simulink model "powertrain_model"  (R2025a)
settings: Solver=ode23tb  StartTime=0.0  StopTime=simlength  FixedStep=tc  MaxStep=tc
values from neighbouring files (symbols this model uses):
  angle_error = angle_error_deg/180*pi    (= 0)    [init_model.m]
  CTRPIFF_CLIP_RELEASE = 0.001    [init_model.m]
  dead_time = dead_time_INV    (= 4.2e-07)    [init_model.m]
  dead_time_INV = 0.42e-6    (= 4.2e-07)    [init_model.m]
  DThs_init = 0    [init_model.m]
  emf_fb_p = 0.2    [init_model.m]
  emf_fb_p_ccaller_1 = emf_fb_p    (= 0.2)    [init_model.m]
  emf_fb_p_ccaller_2 = emf_fb_p    (= 0.2)    [init_model.m]
  emf_p = emf_fb_p*4/10    (= 0.08)    [init_model.m]
  emf_p_ccaller_1 = emf_fb_p_ccaller_1*4/10    (= 0.08)    [init_model.m]
  emf_p_ccaller_2 = emf_fb_p_ccaller_2*4/10    (= 0.08)    [init_model.m]
  fPWM_INV = 25e3    (= 25000)    [init_model.m]
  g0_reference_flt = fcut_reference_flt * ts_inv * 2*pi    (= 0.00100530964915)    [init_model.m]
  g1_reference_flt = 1 - g0_reference_flt    (= 0.998994690351)    [init_model.m]
  id_ref_if_pu = iload_rms_ref*sqrt(2)/ibez    [init_model.m]
  kalman_omega = kw    [init_model.m]
  kalman_theta = kg    [init_model.m]
  kg = K(1)    [init_model.m]
  ki_id = 2    [analysis_cc.m]    (also in init_model.m = 9)
  ki_iq = 9    [init_model.m]
  ki_w = 1    [init_model.m]
  kp_id = 0.15    [analysis_cc.m]    (also in init_model.m = 0.25)
  kp_iq = 0.2    [init_model.m]
  kp_w = 1    [init_model.m]
  kw = K(2)    [init_model.m]
  luenberger_l1 = Klo(1)    [init_model.m]
  luenberger_l2 = Klo(2)    [init_model.m]
  luenberger_l3 = Klo(3)    [init_model.m]
  motorc_m_scale = 2/3*Vdc_bez/ubez    [init_model.m]
  number_of_cells = 100    [init_model.m]
  omega_flt_fcut = 10    [init_model.m]
  omega_flt_g0 = omega_flt_fcut * ts_inv * 2*pi    (= 0.00251327412287)    [init_model.m]
  omega_flt_g1 = 1 - omega_flt_g0    (= 0.997486725877)    [init_model.m]
  omega_ref_if_pu = 1200*2*pi/omega_bez    [init_model.m]
  phase_compensation_omega = 0    [init_model.m]
  pwm_out_lim = 1    [init_model.m]
  Q = 10    [init_model.m]
  q1Kalman = ts_inv^2    (= 1.6e-09)    [init_model.m]
  q2Kalman = ts_inv^1    (= 4e-05)    [init_model.m]
  q3Kalman = 0    [init_model.m]
  rKalman = 1    [init_model.m]
  Tambient = 1    [init_model.m]
  tc = ts_inv/200    (= 2e-07)    [init_model.m]
  time_init = 0.025    [init_model.m]
  torque_ref = 64/ibez*torque_mode    [init_model.m]
  ts_inv = 1/fPWM_INV    (= 4e-05)    [init_model.m]
  tsample = ts_inv    (= 4e-05)    [init_model.m]
  u_flt_g0 = u_flt_fcut * ts_inv * 2*pi    (= 0.904778684234)    [init_model.m]
  u_flt_g1 = 1 - u_flt_g0    (= 0.0952213157661)    [init_model.m]
  Vdc_bez = 400    [init_model.m]
undefined symbols (not defined in the file or in its folder): b, ibez, Jm, Jm_norm, Ld_norm, Lq_norm, Ls_norm, magnitude, omega_bez, psi_bez, psi_m, psi_m_norm, R_RLload, Rload_eq, Rs_norm, tau_bez, weigth
libraries: fl_lib x100, nesl_utility x84, ee_lib x11, cstblocks x4, lithium_ion_cell_lib x1, simulink x1, pmsm_uvw_with_harmonics_lib x1, pmsm_spatial_harmonics_uvw_lib x1, flexshaft_lib x1
(part 2 of 6)

== system powertrain_model/inverter/MOS based inverter ==
  uab : Inport
  Demux : Demux  Outputs=6
  inverter : Subsystem
  sv_pwm : Subsystem
  threePhsModulator : Subsystem  Commented=on
  u : PMIOPort  Side=Left
  v : PMIOPort  Port=2  Side=Left
  w : PMIOPort  Port=3  Side=Left
  UDC(+) : PMIOPort  Port=4  Side=Right
  UDC(-) : PMIOPort  Port=5  Side=Right
  tag scope: gm1=global, gm2=global, gm3=global, gm4=global, gm5=global, gm6=global
  wires:
  Demux/6 -> [gm6]
  Demux/4 -> [gm4]
  Demux/5 -> [gm5]
  Demux/3 -> [gm3]
  Demux/1 -> [gm1]
  Demux/2 -> [gm2]
  sv_pwm/1(firing_gates) -> Demux/1
  uab/1 -> sv_pwm/1(ab), threePhsModulator/1(uab_pu)
  connections:
  inverter/LConn1 -- UDC(+)/RConn1
  inverter/LConn2 -- UDC(-)/RConn1
  v/RConn1 -- inverter/RConn2
  inverter/RConn1 -- u/RConn1
  inverter/RConn3 -- w/RConn1

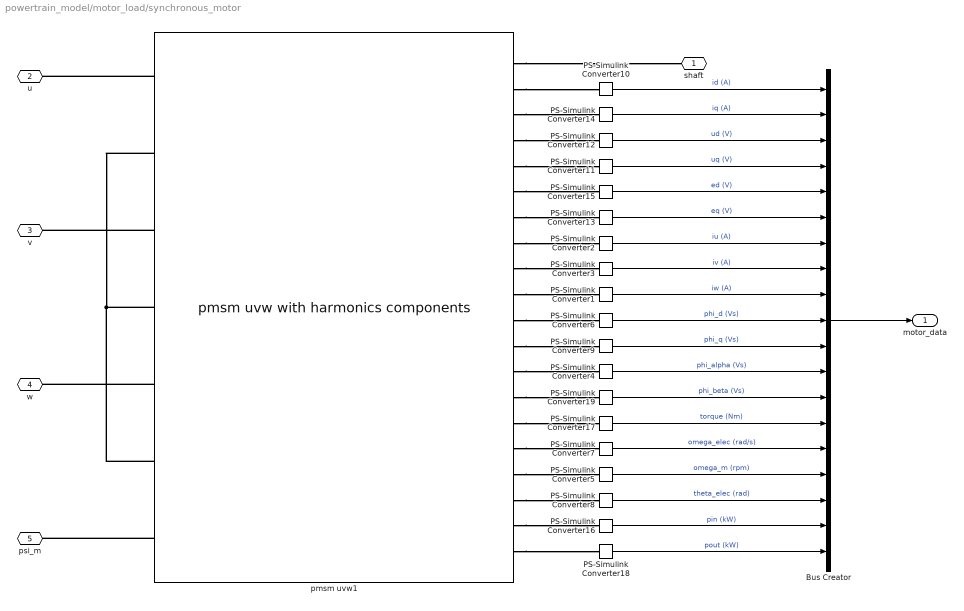
== system powertrain_model/motor_load/synchronous_motor ==
  Bus Creator : BusCreator  Inputs=19
  PS-Simulink Converter1 : nesl_utility/PS-Simulink Converter  PhysicalDomain=network_engine_domain  SubClassName=ps_output  LeftPortType=input  RightPortType=output  PseudoPeriodic=off  Frequencies=[]  VectorFormat=1-D array  Unit=A  AffineConversion=off
  PS-Simulink Converter10 : nesl_utility/PS-Simulink Converter  PhysicalDomain=network_engine_domain  SubClassName=ps_output  LeftPortType=input  RightPortType=output  PseudoPeriodic=off  Frequencies=[]  VectorFormat=1-D array  Unit=A  AffineConversion=on
  PS-Simulink Converter{11..13,15} (4 alike) : nesl_utility/PS-Simulink Converter  PhysicalDomain=network_engine_domain  SubClassName=ps_output  LeftPortType=input  RightPortType=output  PseudoPeriodic=off  Frequencies=[]  VectorFormat=1-D array  Unit=V  AffineConversion=on
  PS-Simulink Converter14 : nesl_utility/PS-Simulink Converter  PhysicalDomain=network_engine_domain  SubClassName=ps_output  LeftPortType=input  RightPortType=output  PseudoPeriodic=off  Frequencies=[]  VectorFormat=1-D array  Unit=A  AffineConversion=on
  PS-Simulink Converter16 : nesl_utility/PS-Simulink Converter  PhysicalDomain=network_engine_domain  SubClassName=ps_output  LeftPortType=input  RightPortType=output  PseudoPeriodic=off  Frequencies=[]  VectorFormat=1-D array  Unit=kW  AffineConversion=on
  PS-Simulink Converter17 : nesl_utility/PS-Simulink Converter  PhysicalDomain=network_engine_domain  SubClassName=ps_output  LeftPortType=input  RightPortType=output  PseudoPeriodic=off  Frequencies=[]  VectorFormat=1-D array  Unit=N*m  AffineConversion=on
  PS-Simulink Converter18 : nesl_utility/PS-Simulink Converter  PhysicalDomain=network_engine_domain  SubClassName=ps_output  LeftPortType=input  RightPortType=output  PseudoPeriodic=off  Frequencies=[]  VectorFormat=1-D array  Unit=kW  AffineConversion=on
  PS-Simulink Converter{4,6,9,19} (4 alike) : nesl_utility/PS-Simulink Converter  PhysicalDomain=network_engine_domain  SubClassName=ps_output  LeftPortType=input  RightPortType=output  PseudoPeriodic=off  Frequencies=[]  VectorFormat=1-D array  Unit=V*s  AffineConversion=on
  PS-Simulink Converter2 : nesl_utility/PS-Simulink Converter  PhysicalDomain=network_engine_domain  SubClassName=ps_output  LeftPortType=input  RightPortType=output  PseudoPeriodic=off  Frequencies=[]  VectorFormat=1-D array  Unit=A  AffineConversion=on
  PS-Simulink Converter3 : nesl_utility/PS-Simulink Converter  PhysicalDomain=network_engine_domain  SubClassName=ps_output  LeftPortType=input  RightPortType=output  PseudoPeriodic=off  Frequencies=[]  VectorFormat=1-D array  Unit=A  AffineConversion=off
  PS-Simulink Converter5 : nesl_utility/PS-Simulink Converter  PhysicalDomain=network_engine_domain  SubClassName=ps_output  LeftPortType=input  RightPortType=output  PseudoPeriodic=off  Frequencies=[]  VectorFormat=1-D array  Unit=rpm  AffineConversion=on
  PS-Simulink Converter7 : nesl_utility/PS-Simulink Converter  PhysicalDomain=network_engine_domain  SubClassName=ps_output  LeftPortType=input  RightPortType=output  PseudoPeriodic=off  Frequencies=[]  VectorFormat=1-D array  Unit=rad/s  AffineConversion=on
  PS-Simulink Converter8 : nesl_utility/PS-Simulink Converter  PhysicalDomain=network_engine_domain  SubClassName=ps_output  LeftPortType=input  RightPortType=output  PseudoPeriodic=off  Frequencies=[]  VectorFormat=1-D array  Unit=rad  AffineConversion=on
  pmsm uvw1 : pmsm_uvw_with_harmonics_lib/pmsm uvw with harmonics components  number_poles=number_poles  psi_m_p=psi_m V*s  Lmu=Lmu H  La=La H  Lb=Lb H  Rs=Rs Ohm  J=Jm kg*m^2  b=0 N*m*s/rad  b_square=0 N*m*s^2/rad^2  h5=4.0 percent  h7=1.0 percent  angle_error=0.5 rad  omega_specify=off  omega_priority=None  omega=0 rad/s  omega_nominal_specify=off  omega_nominal_unit=rad/s  omega_nominal_value=1  theta_specify=off  theta_priority=None  theta=0 rad  theta_nominal_specify=off  theta_nominal_unit=rad  theta_nominal_value=1  iu_specify=off  iu_priority=None  iu=0 A  iu_nominal_specify=off  iu_nominal_unit=A  iu_nominal_value=1  iv_specify=off  iv_priority=None  iv=0 A  iv_nominal_specify=off  iv_nominal_unit=A  iv_nominal_value=1  iw_specify=off  iw_priority=None  iw=0 A  iw_nominal_specify=off  iw_nominal_unit=A  iw_nominal_value=1  id_specify=off  id_priority=None  id=0 A  id_nominal_specify=off  id_nominal_unit=A  id_nominal_value=1  iq_specify=off  iq_priority=None  iq=0 A  iq_nominal_specify=off  iq_nominal_unit=A  iq_nominal_value=1  uv_specify=off  uv_priority=None  uv=0 V  uv_nominal_specify=off  uv_nominal_unit=V  uv_nominal_value=1  uu_specify=off  uu_priority=None  uu=0 V  uu_nominal_specify=off  uu_nominal_unit=V  uu_nominal_value=1  uw_specify=off  uw_priority=None  uw=0 V  uw_nominal_specify=off  uw_nominal_unit=V  uw_nominal_value=1  ud_specify=off  ud_priority=None  ud=0 V  ud_nominal_specify=off  ud_nominal_unit=V  ud_nominal_value=1  uq_specify=off  uq_priority=None  uq=0 V  uq_nominal_specify=off  uq_nominal_unit=V  uq_nominal_value=1  psi_r_u_specify=off  psi_r_u_priority=None  psi_r_u=0 V*s  psi_r_u_nominal_specify=off  psi_r_u_nominal_unit=V*s  psi_r_u_nominal_value=1  psi_r_v_specify=off  psi_r_v_priority=None  psi_r_v=0 V*s  psi_r_v_nominal_specify=off  psi_r_v_nominal_unit=V*s  psi_r_v_nominal_value=1  psi_r_w_specify=off  psi_r_w_priority=None  psi_r_w=0 V*s  psi_r_w_nominal_specify=off  psi_r_w_nominal_unit=V*s  psi_r_w_nominal_value=1  psi_s_d_specify=off  psi_s_d_priority=None  psi_s_d=0.0 V*s  psi_s_d_nominal_specify=off  psi_s_d_nominal_unit=V*s  psi_s_d_nominal_value=1  psi_s_q_specify=off  psi_s_q_priority=None  psi_s_q=0.0 V*s  psi_s_q_nominal_specify=off  psi_s_q_nominal_unit=V*s  psi_s_q_nominal_value=1  psi_r_d_specify=off  psi_r_d_priority=None  psi_r_d=0.0 V*s  psi_r_d_nominal_specify=off  psi_r_d_nominal_unit=V*s  psi_r_d_nominal_value=1  psi_r_q_specify=off  psi_r_q_priority=None  psi_r_q=0.0 V*s  psi_r_q_nominal_specify=off  psi_r_q_nominal_unit=V*s  psi_r_q_nominal_value=1  psi_r_alpha_specify=off  psi_r_alpha_priority=None  psi_r_alpha=0.0 V*s  psi_r_alpha_nominal_specify=off  psi_r_alpha_nominal_unit=V*s  psi_r_alpha_nominal_value=1  psi_r_beta_specify=off  psi_r_beta_priority=None  psi_r_beta=0.0 V*s  psi_r_beta_nominal_specify=off  psi_r_beta_nominal_unit=V*s  psi_r_beta_nominal_value=1  psi_s_alpha_specify=off  psi_s_alpha_priority=None  psi_s_alpha=0.0 V*s  psi_s_alpha_nominal_specify=off  psi_s_alpha_nominal_unit=V*s  psi_s_alpha_nominal_value=1  psi_s_beta_specify=off  psi_s_beta_priority=None  psi_s_beta=0.0 V*s  psi_s_beta_nominal_specify=off  psi_s_beta_nominal_unit=V*s  psi_s_beta_nominal_value=1  tau_l_specify=off  tau_l_priority=None  tau_l=0 N*m  tau_l_nominal_specify=off  tau_l_nominal_unit=N*m  tau_l_nominal_value=1  tau_m_specify=off  tau_m_priority=None  tau_m=0 N*m  tau_m_nominal_specify=off  tau_m_nominal_unit=N*m  tau_m_nominal_value=1
      settings: InternalSimscapePortConfiguration="{\"Bottom\":[],\"Left\":[{\"id\":\"uu_p\",\"label\":\"_uu+_\",\"type\":\"foundation.electrical.electrical\"},{\"id\":\"uu_n\",\"label\":\"_uu-_\",\"type\":\"foundation.electrical.electrical\"},{\"id\":\"uv_p\",\"label\":\"_uv+_\",\"type\":\"foundation.electrical.electrical\"},{\"id\":\"uv_n\",\"label\":\"_uv-_\",\"type\":\"foundation.electrical.electrical\"},{\"id\":\"uw_p\",\"label\":\"_uw+_\",\"type\":\"foundation.electrical.electrical\"},{\"id\":\"uw_n\",\"label\":\"_uw-_\",\"type\":\"foundation.electrical.electrical\"},{\"id\":\"psi_m\",\"label\":\"_psi_m_\",\"type\":\"input\"}],\"Right\":[{\"id\":\"S\",\"label\":\"_S_\",\"type\":\"foundation.mechanical.rotational.rotational\"},{\"id\":\"id_out\",\"label\":\"_id_\",\"type\":\"output\"},{\"id\":\"iq_out\",\"label\":\"_iq_\",\"type\":\"output\"},{\"id\":\"ud_out\",\"label\":\"_ud_\",\"type\":\"output\"},{\"id\":\"uq_out\",\"label\":\"_uq_\",\"type\":\"output\"},{\"id\":\"ed_out\",\"label\":\"_ed_\",\"type\":\"output\"},{\"id\":\"eq_out\",\"label\":\"_eq_\",\"type\":\"output\"},{\"id\":\"iu_out\",\"label\":\"_iu_\",\"type\":\"output\"},{\"id\":\"iv_out\",\"label\":\"_iv_\",\"type\":\"output\"},{\"id\":\"iw_out\",\"label\":\"_iw_\",\"type\":\"output\"},{\"id\":\"psi_r_d_out\",\"label\":\"_psi_r_d_\",\"type\":\"output\"},{\"id\":\"psi_r_q_out\",\"label\":\"_psi_r_q\",\"type\":\"output\"},{\"id\":\"psi_r_alpha_out\",\"label\":\"_psi_r_alpha_\",\"type\":\"output\"},{\"id\":\"psi_r_beta_out\",\"label\":\"_psi_r_beta\",\"type\":\"output\"},{\"id\":\"tau_out\",\"label\":\"_torque_\",\"type\":\"output\"},{\"id\":\"omega_out\",\"label\":\"_omega_elec_\",\"type\":\"output\"},{\"id\":\"omega_m_out\",\"label\":\"_omega_m_\",\"type\":\"output\"},{\"id\":\"theta_out\",\"label\":\"_theta_elec_\",\"type\":\"output\"},{\"id\":\"pin_out\",\"label\":\"_pin_\",\"type\":\"output\"},{\"id\":\"pout_out\",\"label\":\"_pout_\",\"type\":\"output\"}],\"Top\":[]}"
  shaft : PMIOPort  Side=Right
  u : PMIOPort  Port=2  Side=Left
  v : PMIOPort  Port=3  Side=Left
  w : PMIOPort  Port=4  Side=Left
  psi_m : PMIOPort  Port=5  Side=Left
  motor_data : Outport
  wires:
  PS-Simulink Converter10/1 -> Bus Creator/1  "id (A)"
  PS-Simulink Converter14/1 -> Bus Creator/2  "iq (A)"
  PS-Simulink Converter12/1 -> Bus Creator/3  "ud (V)"
  PS-Simulink Converter11/1 -> Bus Creator/4  "uq (V)"
  PS-Simulink Converter15/1 -> Bus Creator/5  "ed (V)"
  PS-Simulink Converter13/1 -> Bus Creator/6  "eq (V)"
  PS-Simulink Converter2/1 -> Bus Creator/7  "iu (A)"
  PS-Simulink Converter3/1 -> Bus Creator/8  "iv (A)"
  PS-Simulink Converter1/1 -> Bus Creator/9  "iw (A)"
  PS-Simulink Converter6/1 -> Bus Creator/10  "phi_d (Vs)"
  PS-Simulink Converter9/1 -> Bus Creator/11  "phi_q (Vs)"
  Bus Creator/1 -> motor_data/1
  PS-Simulink Converter18/1 -> Bus Creator/19  "pout (kW)"
  PS-Simulink Converter16/1 -> Bus Creator/18  "pin (kW)"
  PS-Simulink Converter8/1 -> Bus Creator/17  "theta_elec (rad)"
  PS-Simulink Converter5/1 -> Bus Creator/16  "omega_m (rpm)"
  PS-Simulink Converter7/1 -> Bus Creator/15  "omega_elec (rad/s)"
  PS-Simulink Converter17/1 -> Bus Creator/14  "torque (Nm)"
  PS-Simulink Converter4/1 -> Bus Creator/12  "phi_alpha (Vs)"
  PS-Simulink Converter19/1 -> Bus Creator/13  "phi_beta (Vs)"
  connections:
  pmsm uvw1/RConn8 -- PS-Simulink Converter2/LConn1
  pmsm uvw1/RConn9 -- PS-Simulink Converter3/LConn1
  pmsm uvw1/RConn3 -- PS-Simulink Converter14/LConn1
  pmsm uvw1/RConn4 -- PS-Simulink Converter12/LConn1
  pmsm uvw1/RConn2 -- PS-Simulink Converter10/LConn1
  pmsm uvw1/LConn2 -- pmsm uvw1/LConn6 -- pmsm uvw1/LConn4
  pmsm uvw1/RConn7 -- PS-Simulink Converter13/LConn1
  pmsm uvw1/LConn1 -- u/RConn1
  pmsm uvw1/RConn12 -- PS-Simulink Converter9/LConn1
  pmsm uvw1/RConn10 -- PS-Simulink Converter1/LConn1
  pmsm uvw1/LConn5 -- w/RConn1
  pmsm uvw1/LConn7 -- psi_m/RConn1
  pmsm uvw1/RConn5 -- PS-Simulink Converter11/LConn1
  pmsm uvw1/RConn11 -- PS-Simulink Converter6/LConn1
  pmsm uvw1/RConn6 -- PS-Simulink Converter15/LConn1
  pmsm uvw1/LConn3 -- v/RConn1
  pmsm uvw1/RConn1 -- shaft/RConn1
  pmsm uvw1/RConn15 -- PS-Simulink Converter17/LConn1
  pmsm uvw1/RConn16 -- PS-Simulink Converter7/LConn1
  pmsm uvw1/RConn17 -- PS-Simulink Converter5/LConn1
  pmsm uvw1/RConn18 -- PS-Simulink Converter8/LConn1
  pmsm uvw1/RConn19 -- PS-Simulink Converter16/LConn1
  pmsm uvw1/RConn20 -- PS-Simulink Converter18/LConn1
  pmsm uvw1/RConn13 -- PS-Simulink Converter4/LConn1
  pmsm uvw1/RConn14 -- PS-Simulink Converter19/LConn1

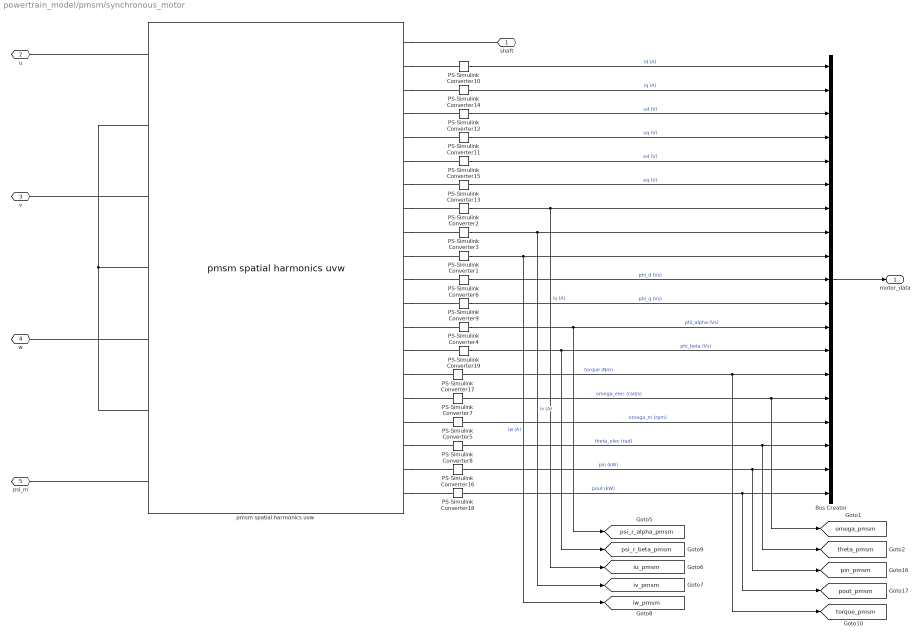
== system powertrain_model/pmsm/synchronous_motor ==
  Bus Creator : BusCreator  Inputs=19
  PS-Simulink Converter{1..3,10,14} (5 alike) : nesl_utility/PS-Simulink Converter  PhysicalDomain=network_engine_domain  SubClassName=ps_output  LeftPortType=input  RightPortType=output  PseudoPeriodic=off  Frequencies=[]  VectorFormat=1-D array  Unit=A  AffineConversion=on
  PS-Simulink Converter{11..13,15} (4 alike) : nesl_utility/PS-Simulink Converter  PhysicalDomain=network_engine_domain  SubClassName=ps_output  LeftPortType=input  RightPortType=output  PseudoPeriodic=off  Frequencies=[]  VectorFormat=1-D array  Unit=V  AffineConversion=on
  PS-Simulink Converter16 : nesl_utility/PS-Simulink Converter  PhysicalDomain=network_engine_domain  SubClassName=ps_output  LeftPortType=input  RightPortType=output  PseudoPeriodic=off  Frequencies=[]  VectorFormat=1-D array  Unit=kW  AffineConversion=on
  PS-Simulink Converter17 : nesl_utility/PS-Simulink Converter  PhysicalDomain=network_engine_domain  SubClassName=ps_output  LeftPortType=input  RightPortType=output  PseudoPeriodic=off  Frequencies=[]  VectorFormat=1-D array  Unit=N*m  AffineConversion=on
  PS-Simulink Converter18 : nesl_utility/PS-Simulink Converter  PhysicalDomain=network_engine_domain  SubClassName=ps_output  LeftPortType=input  RightPortType=output  PseudoPeriodic=off  Frequencies=[]  VectorFormat=1-D array  Unit=kW  AffineConversion=on
  PS-Simulink Converter{4,6,9,19} (4 alike) : nesl_utility/PS-Simulink Converter  PhysicalDomain=network_engine_domain  SubClassName=ps_output  LeftPortType=input  RightPortType=output  PseudoPeriodic=off  Frequencies=[]  VectorFormat=1-D array  Unit=V*s  AffineConversion=on
  PS-Simulink Converter5 : nesl_utility/PS-Simulink Converter  PhysicalDomain=network_engine_domain  SubClassName=ps_output  LeftPortType=input  RightPortType=output  PseudoPeriodic=off  Frequencies=[]  VectorFormat=1-D array  Unit=rpm  AffineConversion=on
  PS-Simulink Converter7 : nesl_utility/PS-Simulink Converter  PhysicalDomain=network_engine_domain  SubClassName=ps_output  LeftPortType=input  RightPortType=output  PseudoPeriodic=off  Frequencies=[]  VectorFormat=1-D array  Unit=rad/s  AffineConversion=on
  PS-Simulink Converter8 : nesl_utility/PS-Simulink Converter  PhysicalDomain=network_engine_domain  SubClassName=ps_output  LeftPortType=input  RightPortType=output  PseudoPeriodic=off  Frequencies=[]  VectorFormat=1-D array  Unit=rad  AffineConversion=on
  pmsm spatial harmonics uvw : pmsm_spatial_harmonics_uvw_lib/pmsm spatial harmonics uvw  number_poles=number_poles  psi_m_p=psi_m V*s  Lmu=Lmu H  La=La H  Lb=Lb H  Rs=Rs Ohm  J=Jm kg*m^2  b=b N*m/(rad/s)  b_square=0 N*m*s^2/rad^2  h5=0 %h5_psm_percent percent  h7=0 %h7_psm_percent percent  omega_specify=off  omega_priority=None  omega=0 rad/s  omega_nominal_specify=off  omega_nominal_unit=rad/s  omega_nominal_value=1  theta_specify=off  theta_priority=None  theta=0 rad  theta_nominal_specify=off  theta_nominal_unit=rad  theta_nominal_value=1  iu_specify=off  iu_priority=None  iu=0 A  iu_nominal_specify=off  iu_nominal_unit=A  iu_nominal_value=1  iv_specify=off  iv_priority=None  iv=0 A  iv_nominal_specify=off  iv_nominal_unit=A  iv_nominal_value=1  iw_specify=off  iw_priority=None  iw=0 A  iw_nominal_specify=off  iw_nominal_unit=A  iw_nominal_value=1  id_specify=off  id_priority=None  id=0 A  id_nominal_specify=off  id_nominal_unit=A  id_nominal_value=1  iq_specify=off  iq_priority=None  iq=0 A  iq_nominal_specify=off  iq_nominal_unit=A  iq_nominal_value=1  uv_specify=off  uv_priority=None  uv=0 V  uv_nominal_specify=off  uv_nominal_unit=V  uv_nominal_value=1  uu_specify=off  uu_priority=None  uu=0 V  uu_nominal_specify=off  uu_nominal_unit=V  uu_nominal_value=1  uw_specify=off  uw_priority=None  uw=0 V  uw_nominal_specify=off  uw_nominal_unit=V  uw_nominal_value=1  ud_specify=off  ud_priority=None  ud=0 V  ud_nominal_specify=off  ud_nominal_unit=V  ud_nominal_value=1  uq_specify=off  uq_priority=None  uq=0 V  uq_nominal_specify=off  uq_nominal_unit=V  uq_nominal_value=1  psi_r_u_specify=off  psi_r_u_priority=None  psi_r_u=0 V*s  psi_r_u_nominal_specify=off  psi_r_u_nominal_unit=V*s  psi_r_u_nominal_value=1  psi_r_v_specify=off  psi_r_v_priority=None  psi_r_v=0 V*s  psi_r_v_nominal_specify=off  psi_r_v_nominal_unit=V*s  psi_r_v_nominal_value=1  psi_r_w_specify=off  psi_r_w_priority=None  psi_r_w=0 V*s  psi_r_w_nominal_specify=off  psi_r_w_nominal_unit=V*s  psi_r_w_nominal_value=1  psi_s_d_specify=off  psi_s_d_priority=None  psi_s_d=0.0 V*s  psi_s_d_nominal_specify=off  psi_s_d_nominal_unit=V*s  psi_s_d_nominal_value=1  psi_s_q_specify=off  psi_s_q_priority=None  psi_s_q=0.0 V*s  psi_s_q_nominal_specify=off  psi_s_q_nominal_unit=V*s  psi_s_q_nominal_value=1  psi_r_d_specify=off  psi_r_d_priority=None  psi_r_d=0.0 V*s  psi_r_d_nominal_specify=off  psi_r_d_nominal_unit=V*s  psi_r_d_nominal_value=1  psi_r_q_specify=off  psi_r_q_priority=None  psi_r_q=0.0 V*s  psi_r_q_nominal_specify=off  psi_r_q_nominal_unit=V*s  psi_r_q_nominal_value=1  psi_r_alpha_specify=on  psi_r_alpha_priority=High  psi_r_alpha=psi_m V*s  psi_r_alpha_nominal_specify=off  psi_r_alpha_nominal_unit=V*s  psi_r_alpha_nominal_value=1  psi_r_beta_specify=on  psi_r_beta_priority=High  psi_r_beta=0.0 V*s  psi_r_beta_nominal_specify=off  psi_r_beta_nominal_unit=V*s  psi_r_beta_nominal_value=1  psi_s_alpha_specify=on  psi_s_alpha_priority=High  psi_s_alpha=psi_m V*s  psi_s_alpha_nominal_specify=off  psi_s_alpha_nominal_unit=V*s  psi_s_alpha_nominal_value=1  psi_s_beta_specify=on  psi_s_beta_priority=High  psi_s_beta=0.0 V*s  psi_s_beta_nominal_specify=off  psi_s_beta_nominal_unit=V*s  psi_s_beta_nominal_value=1  tau_l_specify=off  tau_l_priority=None  tau_l=0 N*m  tau_l_nominal_specify=off  tau_l_nominal_unit=N*m  tau_l_nominal_value=1  tau_m_specify=off  tau_m_priority=None  tau_m=0 N*m  tau_m_nominal_specify=off  tau_m_nominal_unit=N*m  tau_m_nominal_value=1
      settings: InternalSimscapePortConfiguration="{\"Bottom\":[],\"Left\":[{\"id\":\"uu_p\",\"label\":\"_uu+_\",\"type\":\"foundation.electrical.electrical\"},{\"id\":\"uu_n\",\"label\":\"_uu-_\",\"type\":\"foundation.electrical.electrical\"},{\"id\":\"uv_p\",\"label\":\"_uv+_\",\"type\":\"foundation.electrical.electrical\"},{\"id\":\"uv_n\",\"label\":\"_uv-_\",\"type\":\"foundation.electrical.electrical\"},{\"id\":\"uw_p\",\"label\":\"_uw+_\",\"type\":\"foundation.electrical.electrical\"},{\"id\":\"uw_n\",\"label\":\"_uw-_\",\"type\":\"foundation.electrical.electrical\"},{\"id\":\"psi_m\",\"label\":\"_psi_m_\",\"type\":\"input\"}],\"Right\":[{\"id\":\"S\",\"label\":\"_S_\",\"type\":\"foundation.mechanical.rotational.rotational\"},{\"id\":\"id_out\",\"label\":\"_id_\",\"type\":\"output\"},{\"id\":\"iq_out\",\"label\":\"_iq_\",\"type\":\"output\"},{\"id\":\"ud_out\",\"label\":\"_ud_\",\"type\":\"output\"},{\"id\":\"uq_out\",\"label\":\"_uq_\",\"type\":\"output\"},{\"id\":\"ed_out\",\"label\":\"_ed_\",\"type\":\"output\"},{\"id\":\"eq_out\",\"label\":\"_eq_\",\"type\":\"output\"},{\"id\":\"iu_out\",\"label\":\"_iu_\",\"type\":\"output\"},{\"id\":\"iv_out\",\"label\":\"_iv_\",\"type\":\"output\"},{\"id\":\"iw_out\",\"label\":\"_iw_\",\"type\":\"output\"},{\"id\":\"psi_r_d_out\",\"label\":\"_psi_r_d_\",\"type\":\"output\"},{\"id\":\"psi_r_q_out\",\"label\":\"_psi_r_q\",\"type\":\"output\"},{\"id\":\"psi_r_alpha_out\",\"label\":\"_psi_r_alpha_\",\"type\":\"output\"},{\"id\":\"psi_r_beta_out\",\"label\":\"_psi_r_beta\",\"type\":\"output\"},{\"id\":\"tau_out\",\"label\":\"_torque_\",\"type\":\"output\"},{\"id\":\"omega_out\",\"label\":\"_omega_elec_\",\"type\":\"output\"},{\"id\":\"omega_m_out\",\"label\":\"_omega_m_\",\"type\":\"output\"},{\"id\":\"theta_out\",\"label\":\"_theta_elec_\",\"type\":\"output\"},{\"id\":\"pin_out\",\"label\":\"_pin_\",\"type\":\"output\"},{\"id\":\"pout_out\",\"label\":\"_pout_\",\"type\":\"output\"}],\"Top\":[]}"
  shaft : PMIOPort  Side=Right
  u : PMIOPort  Port=2  Side=Left
  v : PMIOPort  Port=3  Side=Left
  w : PMIOPort  Port=4  Side=Left
  psi_m : PMIOPort  Port=5  Side=Left
  motor_data : Outport
  tag scope: iu_pmsm=global, iv_pmsm=global, iw_pmsm=global, omega_pmsm=global, pin_pmsm=global, pout_pmsm=global, psi_r_alpha_pmsm=global, psi_r_beta_pmsm=global, theta_pmsm=global, torque_pmsm=global
  wires:
  PS-Simulink Converter10/1 -> Bus Creator/1  "id (A)"
  PS-Simulink Converter14/1 -> Bus Creator/2  "iq (A)"
  PS-Simulink Converter12/1 -> Bus Creator/3  "ud (V)"
  PS-Simulink Converter11/1 -> Bus Creator/4  "uq (V)"
  PS-Simulink Converter15/1 -> Bus Creator/5  "ed (V)"
  PS-Simulink Converter13/1 -> Bus Creator/6  "eq (V)"
  PS-Simulink Converter2/1 -> Bus Creator/7, [iu_pmsm]  "iu (A)"
  PS-Simulink Converter3/1 -> Bus Creator/8, [iv_pmsm]  "iv (A)"
  PS-Simulink Converter1/1 -> Bus Creator/9, [iw_pmsm]  "iw (A)"
  PS-Simulink Converter6/1 -> Bus Creator/10  "phi_d (Vs)"
  PS-Simulink Converter9/1 -> Bus Creator/11  "phi_q (Vs)"
  Bus Creator/1 -> motor_data/1
  PS-Simulink Converter18/1 -> [pout_pmsm], Bus Creator/19  "pout (kW)"
  PS-Simulink Converter16/1 -> [pin_pmsm], Bus Creator/18  "pin (kW)"
  PS-Simulink Converter8/1 -> [theta_pmsm], Bus Creator/17  "theta_elec (rad)"
  PS-Simulink Converter5/1 -> Bus Creator/16  "omega_m (rpm)"
  PS-Simulink Converter7/1 -> [omega_pmsm], Bus Creator/15  "omega_elec (rad/s)"
  PS-Simulink Converter17/1 -> [torque_pmsm], Bus Creator/14  "torque (Nm)"
  PS-Simulink Converter4/1 -> Bus Creator/12, [psi_r_alpha_pmsm]  "phi_alpha (Vs)"
  PS-Simulink Converter19/1 -> Bus Creator/13, [psi_r_beta_pmsm]  "phi_beta (Vs)"
  connections:
  pmsm spatial harmonics uvw/RConn8 -- PS-Simulink Converter2/LConn1
  pmsm spatial harmonics uvw/RConn9 -- PS-Simulink Converter3/LConn1
  pmsm spatial harmonics uvw/RConn3 -- PS-Simulink Converter14/LConn1
  pmsm spatial harmonics uvw/RConn4 -- PS-Simulink Converter12/LConn1
  pmsm spatial harmonics uvw/RConn2 -- PS-Simulink Converter10/LConn1
  pmsm spatial harmonics uvw/LConn2 -- pmsm spatial harmonics uvw/LConn6 -- pmsm spatial harmonics uvw/LConn4
  pmsm spatial harmonics uvw/RConn7 -- PS-Simulink Converter13/LConn1
  pmsm spatial harmonics uvw/LConn1 -- u/RConn1
  pmsm spatial harmonics uvw/RConn12 -- PS-Simulink Converter9/LConn1
  pmsm spatial harmonics uvw/RConn10 -- PS-Simulink Converter1/LConn1
  pmsm spatial harmonics uvw/LConn5 -- w/RConn1
  pmsm spatial harmonics uvw/LConn7 -- psi_m/RConn1
  pmsm spatial harmonics uvw/RConn5 -- PS-Simulink Converter11/LConn1
  pmsm spatial harmonics uvw/RConn11 -- PS-Simulink Converter6/LConn1
  pmsm spatial harmonics uvw/RConn6 -- PS-Simulink Converter15/LConn1
  pmsm spatial harmonics uvw/LConn3 -- v/RConn1
  pmsm spatial harmonics uvw/RConn1 -- shaft/RConn1
  pmsm spatial harmonics uvw/RConn15 -- PS-Simulink Converter17/LConn1
  pmsm spatial harmonics uvw/RConn16 -- PS-Simulink Converter7/LConn1
  pmsm spatial harmonics uvw/RConn17 -- PS-Simulink Converter5/LConn1
  pmsm spatial harmonics uvw/RConn18 -- PS-Simulink Converter8/LConn1
  pmsm spatial harmonics uvw/RConn19 -- PS-Simulink Converter16/LConn1
  pmsm spatial harmonics uvw/RConn20 -- PS-Simulink Converter18/LConn1
  pmsm spatial harmonics uvw/RConn13 -- PS-Simulink Converter4/LConn1
  pmsm spatial harmonics uvw/RConn14 -- PS-Simulink Converter19/LConn1

== system powertrain_model/propeller/Subsystem ==
  flexible shaft : flexshaft_lib/flexible shaft  b1=0 N*m*s/rad  J1=1e-4 kg*m^2  b2=0 N*m*s/rad  J2=1e-4 kg*m^2  b_theta=0 N*m*s/rad  k_theta=1e12 N*m/rad  w_1_specify=off  w_1_priority=None  w_1=0 rad/s  w_1_nominal_specify=off  w_1_nominal_value=1  w_1_nominal_unit=rad/s  w_2_specify=off  w_2_priority=None  w_2=0 rad/s  w_2_nominal_specify=off  w_2_nominal_value=1  w_2_nominal_unit=rad/s  t_1_specify=off  t_1_priority=None  t_1=0 N*m  t_1_nominal_specify=off  t_1_nominal_value=1  t_1_nominal_unit=N*m  t_2_specify=off  t_2_priority=None  t_2=0 N*m  t_2_nominal_specify=off  t_2_nominal_value=1  t_2_nominal_unit=N*m  t_theta_specify=off  t_theta_priority=None  t_theta=0 N*m  t_theta_nominal_specify=off  t_theta_nominal_value=1  t_theta_nominal_unit=N*m
      settings: InternalSimscapePortConfiguration="{\"Bottom\":[],\"Left\":[{\"id\":\"S1\",\"label\":\"S1\",\"type\":\"foundation.mechanical.rotational.rotational\"}],\"Right\":[{\"id\":\"S2\",\"label\":\"S2\",\"type\":\"foundation.mechanical.rotational.rotational\"}],\"Top\":[]}"
  s2 : PMIOPort  Side=Right
  s1 : PMIOPort  Port=2  Side=Left
  connections:
  flexible shaft/RConn1 -- s2/RConn1
  flexible shaft/LConn1 -- s1/RConn1

== system powertrain_model/battery_system/battery_system/LithiumIonBattery ==
  Current Sensor : fl_lib/Electrical/Electrical Sensors/Current Sensor
  Electrical Reference1 : fl_lib/Electrical/Electrical Elements/Electrical Reference
  PS-Simulink Converter4 : nesl_utility/PS-Simulink Converter  PhysicalDomain=network_engine_domain  SubClassName=ps_output  LeftPortType=input  RightPortType=output  PseudoPeriodic=off  Frequencies=[]  VectorFormat=1-D array  Unit=1  AffineConversion=off
  PS-Simulink Converter5 : nesl_utility/PS-Simulink Converter  PhysicalDomain=network_engine_domain  SubClassName=ps_output  LeftPortType=input  RightPortType=output  PseudoPeriodic=off  Frequencies=[]  VectorFormat=1-D array  Unit=V  AffineConversion=on
  SOC_estimator : Subsystem
  To Workspace1 : ToWorkspace  VariableName=idc_battery_sim  SampleTime=tc
      settings: MaxDataPoints=Nc
  To Workspace2 : ToWorkspace  VariableName=udc_battery_sim  SampleTime=tc
      settings: MaxDataPoints=Nc
  Unit Delay5 : UnitDelay  SampleTime=tsample  HasFrameUpgradeWarning=on
  Voltage Sensor : fl_lib/Electrical/Electrical Sensors/Voltage Sensor
  ibat/vdc : Scope  Commented=on  NumInputPorts=2
      settings: SampleTime=tsample  ActiveDisplayYMinimum=-422.32966  ActiveDisplayYMaximum=499.01489  DataLoggingVariableName=ScopeData6
  lithium ion cell analytical ocv : Subsystem
  Uout+ : PMIOPort  Side=Right
  Uout- : PMIOPort  Port=2  Side=Right
  wires:
  PS-Simulink Converter5/1 -> Unit Delay5/1
  PS-Simulink Converter4/1 -> To Workspace1/1, ibat/vdc/1  "i batt"
  Unit Delay5/1 -> To Workspace2/1, [vdc]
  [vdc] -> ibat/vdc/2  "vdc"
  connections:
  Current Sensor/RConn1 -- PS-Simulink Converter4/LConn1
  Uout+/RConn1 -- Current Sensor/RConn2 -- Voltage Sensor/LConn1
  Voltage Sensor/RConn1 -- PS-Simulink Converter5/LConn1
  Voltage Sensor/RConn2 -- Electrical Reference1/LConn1 -- lithium ion cell analytical ocv/RConn2 -- Uout-/RConn1
  lithium ion cell analytical ocv/RConn1 -- Current Sensor/LConn1

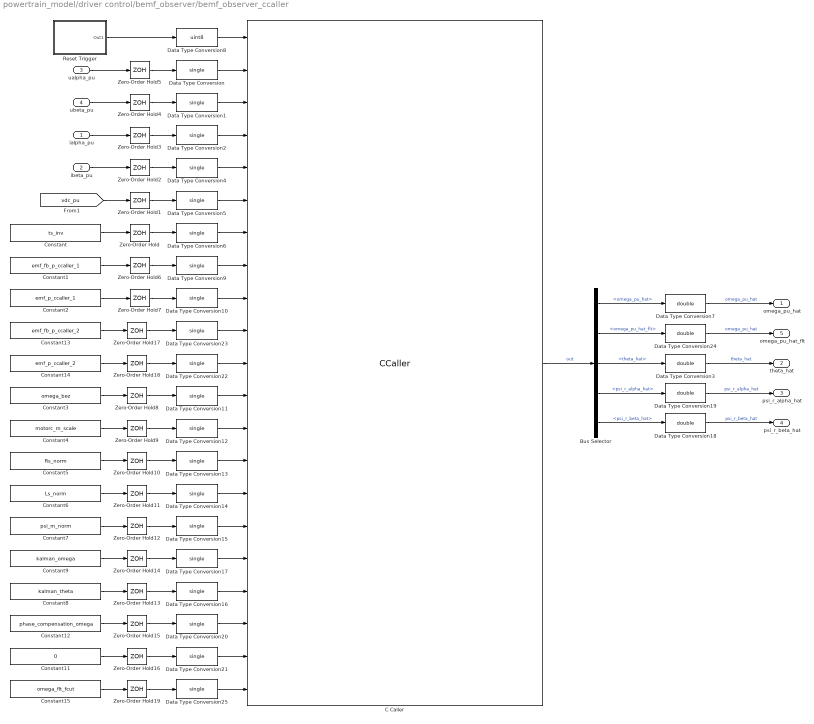
== system powertrain_model/driver control/bemf_observer/bemf_observer_ccaller ==
  ialpha_pu : Inport
  ibeta_pu : Inport  Port=2
  ualpha_pu : Inport  Port=3
  ubeta_pu : Inport  Port=4
  Bus Selector : BusSelector  OutputSignals=omega_pu_hat,omega_pu_hat_flt,theta_hat,psi_r_alpha_hat,psi_r_beta_hat
  C Caller : CCaller  FunctionName=bemf_obsv_process_simulink  PortSpecificationStruct="%)30     .    N\"8   8    (     @         %    \"    !8    !     0         %  0 \"0    $    _    07)G3F%M90  4&]R=$YA;64 4V-O<&4     26YD97@     5'EP90      4VEZ90      27-';&]B86P   X    P    !@    @    $          4    (     0    ,    !         !   P!O=70 #@   #     &    \"     0         !0    @    !     P    $         $  # &]U=  .    .     8    (    !          %    \"     $    &     0         0  ...(+12985 chars)"  SampleTime=ts_inv
  Constant : Constant  Value=ts_inv
  Constant1 : Constant  Value=emf_fb_p_ccaller_1
  Constant11 : Constant  Value=0
  Constant12 : Constant  Value=phase_compensation_omega  VectorParams1D=off
  Constant13 : Constant  Value=emf_fb_p_ccaller_2
  Constant14 : Constant  Value=emf_p_ccaller_2
  Constant15 : Constant  Value=omega_flt_fcut
  Constant2 : Constant  Value=emf_p_ccaller_1
  Constant3 : Constant  Value=omega_bez
  Constant4 : Constant  Value=motorc_m_scale
  Constant5 : Constant  Value=Rs_norm
  Constant6 : Constant  Value=Ls_norm
  Constant7 : Constant  Value=psi_m_norm
  Constant8 : Constant  Value=kalman_theta
  Constant9 : Constant  Value=kalman_omega
  Data Type Conversion{,1..2,4..6,9..17,20..23,25} (20 alike) : DataTypeConversion  OutDataTypeStr=single  SaturateOnIntegerOverflow=off  RndMeth=Floor
  Data Type Conversion{3,7,18..19,24} (5 alike) : DataTypeConversion  OutDataTypeStr=double  SaturateOnIntegerOverflow=off  RndMeth=Floor
  Data Type Conversion8 : DataTypeConversion  OutDataTypeStr=uint8  SaturateOnIntegerOverflow=off  RndMeth=Floor
  Reset Trigger : Subsystem
  Zero-Order Hold{,1..19} (20 alike) : ZeroOrderHold  SampleTime=ts_inv
  omega_pu_hat : Outport
  theta_hat : Outport  Port=2
  psi_r_alpha_hat : Outport  Port=3
  psi_r_beta_hat : Outport  Port=4
  omega_pu_hat_flt : Outport  Port=5
  wires:
  Bus Selector/1 -> Data Type Conversion7/1  "<omega_pu_hat>"
  Bus Selector/2 -> Data Type Conversion24/1  "<omega_pu_hat_flt>"
  Bus Selector/3 -> Data Type Conversion3/1  "<theta_hat>"
  Bus Selector/4 -> Data Type Conversion19/1  "<psi_r_alpha_hat>"
  Bus Selector/5 -> Data Type Conversion18/1  "<psi_r_beta_hat>"
  Zero-Order Hold19/1 -> Data Type Conversion25/1
  Constant15/1 -> Zero-Order Hold19/1
  Data Type Conversion24/1 -> omega_pu_hat_flt/1  "omega_pu_hat"
  Zero-Order Hold17/1 -> Data Type Conversion23/1
  Zero-Order Hold18/1 -> Data Type Conversion22/1
  Constant13/1 -> Zero-Order Hold17/1
  Constant14/1 -> Zero-Order Hold18/1
  Constant11/1 -> Zero-Order Hold16/1
  Zero-Order Hold16/1 -> Data Type Conversion21/1
  Zero-Order Hold15/1 -> Data Type Conversion20/1
  Constant12/1 -> Zero-Order Hold15/1
  Constant2/1 -> Zero-Order Hold7/1
  Constant1/1 -> Zero-Order Hold6/1
  Data Type Conversion18/1 -> psi_r_beta_hat/1  "psi_r_beta_hat"
  Data Type Conversion19/1 -> psi_r_alpha_hat/1  "psi_r_alpha_hat"
  Data Type Conversion3/1 -> theta_hat/1  "theta_hat"
  Data Type Conversion7/1 -> omega_pu_hat/1  "omega_pu_hat"
  C Caller/1 -> Bus Selector/1  "out"
  Constant7/1 -> Zero-Order Hold12/1
  Constant6/1 -> Zero-Order Hold11/1
  Constant9/1 -> Zero-Order Hold14/1
  Constant8/1 -> Zero-Order Hold13/1
  Constant5/1 -> Zero-Order Hold10/1
  Constant4/1 -> Zero-Order Hold9/1
  Constant3/1 -> Zero-Order Hold8/1
  Zero-Order Hold14/1 -> Data Type Conversion17/1
  Zero-Order Hold13/1 -> Data Type Conversion16/1
  Zero-Order Hold12/1 -> Data Type Conversion15/1
  Zero-Order Hold11/1 -> Data Type Conversion14/1
  Zero-Order Hold10/1 -> Data Type Conversion13/1
  Zero-Order Hold9/1 -> Data Type Conversion12/1
  Zero-Order Hold8/1 -> Data Type Conversion11/1
  Zero-Order Hold7/1 -> Data Type Conversion10/1
  Zero-Order Hold6/1 -> Data Type Conversion9/1
  Reset Trigger/1(Out1) -> Data Type Conversion8/1
  ibeta_pu/1 -> Zero-Order Hold2/1
  ubeta_pu/1 -> Zero-Order Hold4/1
  ialpha_pu/1 -> Zero-Order Hold3/1
  ualpha_pu/1 -> Zero-Order Hold5/1
  Constant/1 -> Zero-Order Hold/1
  [vdc_pu] -> Zero-Order Hold1/1
  Zero-Order Hold1/1 -> Data Type Conversion5/1
  Zero-Order Hold2/1 -> Data Type Conversion4/1
  Zero-Order Hold3/1 -> Data Type Conversion2/1
  Zero-Order Hold4/1 -> Data Type Conversion1/1
  Zero-Order Hold5/1 -> Data Type Conversion/1
  Zero-Order Hold/1 -> Data Type Conversion6/1
  Data Type Conversion/1 -> C Caller/2
  Data Type Conversion8/1 -> C Caller/1
  Data Type Conversion1/1 -> C Caller/3
  Data Type Conversion2/1 -> C Caller/4
  Data Type Conversion4/1 -> C Caller/5
  Data Type Conversion5/1 -> C Caller/6
  Data Type Conversion6/1 -> C Caller/7
  Data Type Conversion9/1 -> C Caller/8
  Data Type Conversion10/1 -> C Caller/9
  Data Type Conversion23/1 -> C Caller/10
  Data Type Conversion22/1 -> C Caller/11
  Data Type Conversion11/1 -> C Caller/12
  Data Type Conversion12/1 -> C Caller/13
  Data Type Conversion13/1 -> C Caller/14
  Data Type Conversion14/1 -> C Caller/15
  Data Type Conversion15/1 -> C Caller/16
  Data Type Conversion17/1 -> C Caller/17
  Data Type Conversion16/1 -> C Caller/18
  Data Type Conversion20/1 -> C Caller/19
  Data Type Conversion21/1 -> C Caller/20
  Data Type Conversion25/1 -> C Caller/21
